simulink model "zad3"  (R2022b)
settings: Solver=FixedStepAuto  StartTime=0.0  StopTime=4  FixedStep=0.00001  RelTol=1e-3
model workspace (MAT data in the model file):
  a0 = 1
  a1 = 1
undefined symbols (not defined in the file): Ki, Kp
settings Model: Creator=vandm  LastModifiedBy=vandm

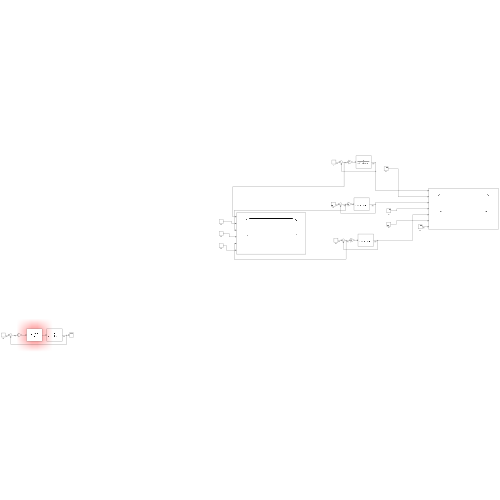
[thumbnail: Simulink's stored preview of the top-level diagram]
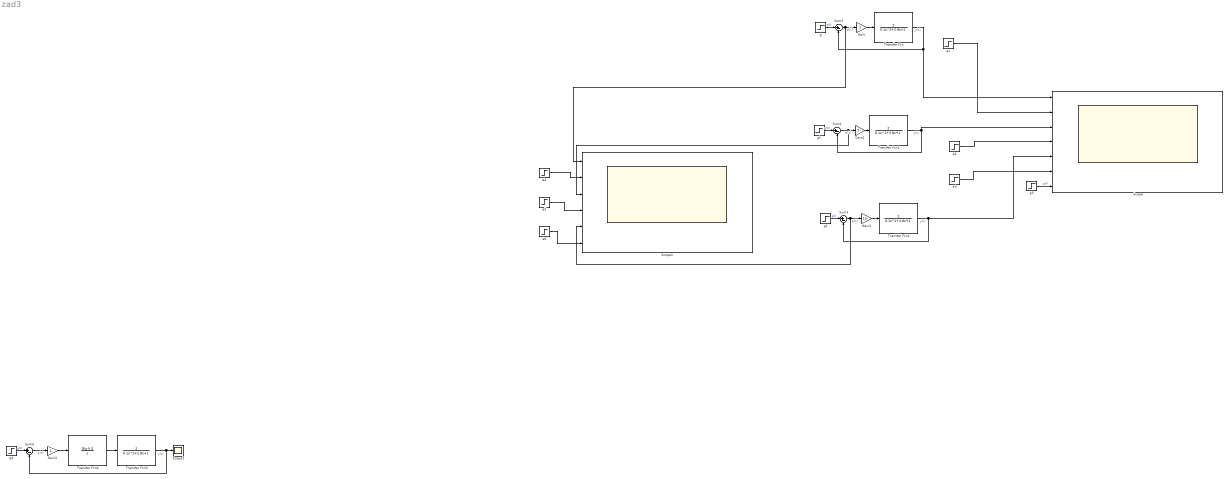
== system zad3 ==
  note: e(t)
  note: y(t)
  note: y(t)
  note: e(t)
  note: y(t)
  note: e(t)
  note: e(t)
  note: y(t)
  Gain : Gain
  Gain1 : Gain  Gain=5
  Gain2 : Gain  Gain=10
  Gain3 : Gain
  Scope : Scope  NumInputPorts=7
  Scope1 : Scope  NumInputPorts=6
  Scope2 : Scope
  Sum{1..4} (4 alike) : Sum  Inputs=|+-
  Transfer Fcn{,1..3} (4 alike) : TransferFcn  Numerator=[2]  Denominator=[0.1 2.8 1]
  Transfer Fcn4 : TransferFcn  Numerator=[Kp Ki]  Denominator=[1 0]
  e1 : Step  Time=0  After=3 - 3/(1 + 2)  SampleTime=0
  e2 : Step  Time=0  After=3 - 3/(1 + 2 * 5)  SampleTime=0
  e3 : Step  Time=0  After=3 - 3/(1 + 2 * 10)  SampleTime=0
  e4 : Step  Time=0  After=3/(1 + 2)  SampleTime=0
  e5 : Step  Time=0  After=3/(1 + 2 * 5)  SampleTime=0
  e6 : Step  Time=0  After=3/(1 + 2 * 10)  SampleTime=0
  g{,1..4} (5 alike) : Step  Time=0  After=3  SampleTime=0
  wires:
  g/1 -> Sum2/1  "g(t)"
  Sum2/1 -> Scope1/1, Gain/1
  Gain/1 -> Transfer Fcn/1
  Transfer Fcn/1 -> Sum2/2, Scope/1
  e1/1 -> Scope/2
  Sum1/1 -> Scope1/3, Gain1/1
  g1/1 -> Sum1/1  "g(t)"
  Gain1/1 -> Transfer Fcn1/1
  Transfer Fcn1/1 -> Scope/3, Sum1/2
  e2/1 -> Scope/4
  Transfer Fcn2/1 -> Scope/5, Sum3/2
  g2/1 -> Sum3/1  "g(t)"
  Gain2/1 -> Transfer Fcn2/1
  Sum3/1 -> Scope1/5, Gain2/1
  e3/1 -> Scope/6
  g3/1 -> Scope/7  "g(t)"
  e4/1 -> Scope1/2
  e5/1 -> Scope1/4
  e6/1 -> Scope1/6
  Sum4/1 -> Gain3/1
  Transfer Fcn3/1 -> Scope2/1, Sum4/2
  g4/1 -> Sum4/1  "g(t)"
  Transfer Fcn4/1 -> Transfer Fcn3/1
  Gain3/1 -> Transfer Fcn4/1
